simulink model "sensorPlantValidation"  (R2026a)
settings: Solver=VariableStepAuto  StopTime=600
values from neighbouring files (symbols this model uses):
  sensorParams = S.sensorParams    [validateFull.m]
undefined symbols (not defined in the file or in its folder): dspblkCoreblockFVToolHelper, gcbh
libraries: simulink x2
settings Model: Creator=ericssonlin  LastModifiedBy=ericssonlin

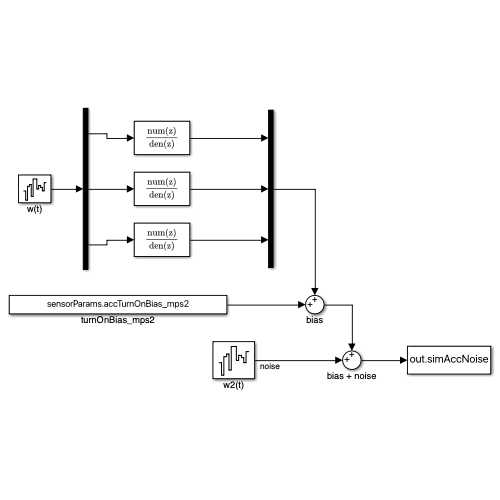
[thumbnail: Simulink's stored preview of the top-level diagram]
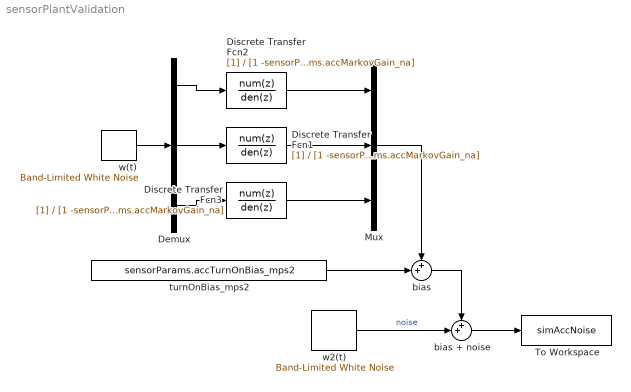
== system sensorPlantValidation ==
  Demux : Demux  Outputs=3
  Discrete Transfer Fcn1 : DiscreteTransferFcn  LoadFcn=dspblkCoreblockFVToolHelper(gcbh,'load');  Denominator=[1 -sensorParams.accMarkovGain_na]
      settings: CopyFcn=dspblkCoreblockFVToolHelper(gcbh,'copy');  DeleteFcn=dspblkCoreblockFVToolHelper(gcbh,'close');  ModelCloseFcn=dspblkCoreblockFVToolHelper(gcbh,'close');  PreSaveFcn=dspblkCoreblockFVToolHelper(gcbh,'presave');  PostSaveFcn=dspblkCoreblockFVToolHelper(gcbh,'postsave');  CloseFcn=dspblkCoreblockFVToolHelper(gcbh,'close');
  Discrete Transfer Fcn2 : DiscreteTransferFcn  LoadFcn=dspblkCoreblockFVToolHelper(gcbh,'load');  Denominator=[1 -sensorParams.accMarkovGain_na]
      settings: CopyFcn=dspblkCoreblockFVToolHelper(gcbh,'copy');  DeleteFcn=dspblkCoreblockFVToolHelper(gcbh,'close');  ModelCloseFcn=dspblkCoreblockFVToolHelper(gcbh,'close');  PreSaveFcn=dspblkCoreblockFVToolHelper(gcbh,'presave');  PostSaveFcn=dspblkCoreblockFVToolHelper(gcbh,'postsave');  CloseFcn=dspblkCoreblockFVToolHelper(gcbh,'close');
  Discrete Transfer Fcn3 : DiscreteTransferFcn  LoadFcn=dspblkCoreblockFVToolHelper(gcbh,'load');  Denominator=[1 -sensorParams.accMarkovGain_na]
      settings: CopyFcn=dspblkCoreblockFVToolHelper(gcbh,'copy');  DeleteFcn=dspblkCoreblockFVToolHelper(gcbh,'close');  ModelCloseFcn=dspblkCoreblockFVToolHelper(gcbh,'close');  PreSaveFcn=dspblkCoreblockFVToolHelper(gcbh,'presave');  PostSaveFcn=dspblkCoreblockFVToolHelper(gcbh,'postsave');  CloseFcn=dspblkCoreblockFVToolHelper(gcbh,'close');
  Mux : Mux  Inputs=3
  To Workspace : ToWorkspace  VariableName=simAccNoise  SaveFormat=Timeseries  SampleTime=-1
  bias : Sum  Inputs=++|
  bias + noise : Sum  Inputs=++|
  turnOnBias_mps2 : Constant  Value=sensorParams.accTurnOnBias_mps2
  w(t) : simulink/Sources/Band-Limited White Noise  Cov=sensorParams.accRWNoisePower  Ts=sensorParams.accSampleTime_s  seed=[101, 202, 303]
  w2(t) : simulink/Sources/Band-Limited White Noise  Cov=sensorParams.accWhiteNoiseStrengths  Ts=sensorParams.accSampleTime_s  seed=[42, 67, 69]
  wires:
  w(t)/1 -> Demux/1
  Demux/2 -> Discrete Transfer Fcn1/1
  Discrete Transfer Fcn1/1 -> Mux/2
  Demux/1 -> Discrete Transfer Fcn2/1
  Discrete Transfer Fcn2/1 -> Mux/1
  Demux/3 -> Discrete Transfer Fcn3/1
  Discrete Transfer Fcn3/1 -> Mux/3
  Mux/1 -> bias/1
  turnOnBias_mps2/1 -> bias/2
  bias/1 -> bias + noise/1
  w2(t)/1 -> bias + noise/2  "noise"
  bias + noise/1 -> To Workspace/1
